simulink model "GRID_SUPPORTED_WIND_R1"  (R2026a)
settings: Solver=ode14x  StopTime=1.1  FixedStep=1e-5
InitFcn:
  | setup_v2_paths; init_grid_supported_integration;
undefined symbols (not defined in the file): Base, Control, Converter, Drive, Filter, PMSG, V2, Wind
libraries: nesl_utility x21, ee_lib x14, fl_lib x6, simulink x1
(part 1 of 2)
Description:
  | PV physical DC + optional corrected Wind R4 averaged GSC integration. The synchronous machine remains connected in every test. No BESS replacement or island certification.
settings Model: Creator=fakebob2004  LastModifiedBy=fakebob2004

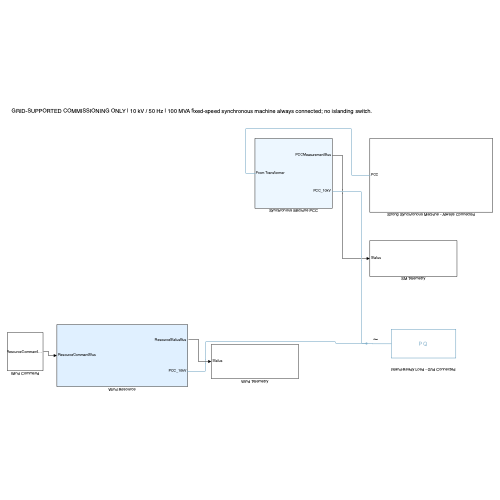
[thumbnail: Simulink's stored preview of the top-level diagram]
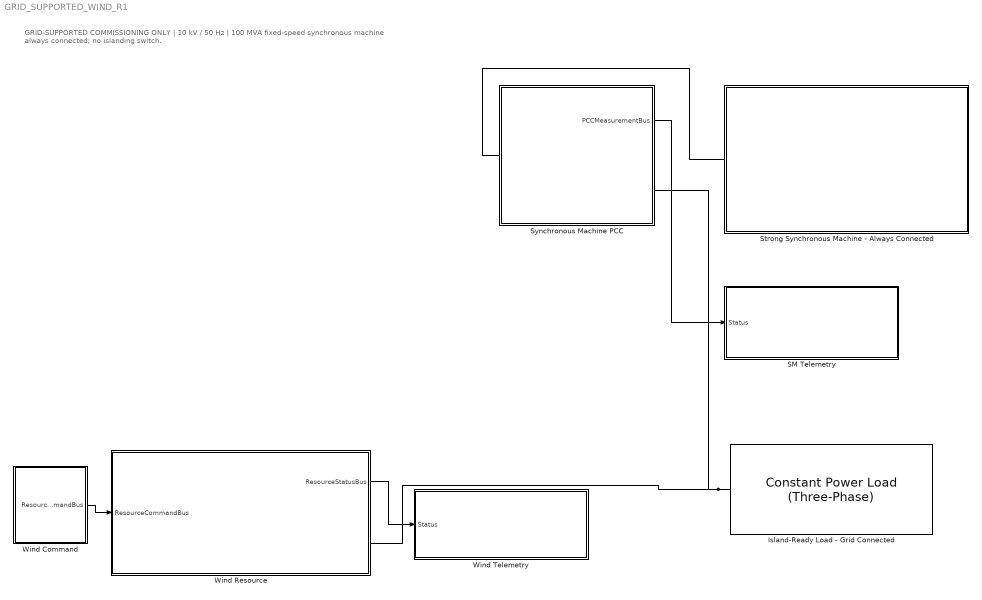
== system GRID_SUPPORTED_WIND_R1 ==
  note: GRID-SUPPORTED COMMISSIONING ONLY | 10 kV / 50 Hz | 100 MVA fixed-speed synchronous machine always connected; no islanding switch.
  Island-Ready Load - Grid Connected : ee_lib/Passive/Constant Power Load (Three-Phase)  port_option=ee.enum.threePhasePort.composite  FRated=50 Hz  active_power=5e6 W  reactive_power=1.5e6 V*A  Vline_rms_min=7000 V  tau=0.01 s  Vline_rms_ini=10000 V  Vang_ini=0 deg  gmin=1e-6 S
  SM Telemetry : Subsystem
  Strong Synchronous Machine - Always Connected : Subsystem
  Synchronous Machine PCC : Subsystem
  Wind Command : Subsystem
  Wind Resource : Subsystem
  Wind Telemetry : Subsystem
  wires:
  Synchronous Machine PCC/1(PCCMeasurementBus) -> SM Telemetry/1(Status)
  Wind Command/1(ResourceCommandBus) -> Wind Resource/1(ResourceCommandBus)
  Wind Resource/1(ResourceStatusBus) -> Wind Telemetry/1(Status)
  connections:
  Strong Synchronous Machine - Always Connected/LConn1 -- Synchronous Machine PCC/LConn1
  Synchronous Machine PCC/RConn1 -- Wind Resource/RConn1 -- Island-Ready Load - Grid Connected/LConn1

== system GRID_SUPPORTED_WIND_R1/SM Telemetry ==
  Status : Inport
  Fields : BusSelector  OutputSignals=P_W,Q_var,Vll_rms_V
  Record : ToWorkspace  VariableName=integration_sm  SaveFormat=Timeseries  SampleTime=-1
  Vector : Mux  Inputs=3
  wires:
  Status/1 -> Fields/1
  Fields/1 -> Vector/1  "<P_W>"
  Fields/2 -> Vector/2  "<Q_var>"
  Fields/3 -> Vector/3  "<Vll_rms_V>"
  Vector/1 -> Record/1

== system GRID_SUPPORTED_WIND_R1/Strong Synchronous Machine - Always Connected ==
  Excitation : Constant  Value=1e4*sqrt(2/3)
  Excitation PS : nesl_utility/Simulink-PS Converter  PhysicalDomain=network_engine_domain  SubClassName=ps_input  LeftPortType=input  RightPortType=output  PseudoPeriodic=off  Frequencies=[]  NoiseDistribution=none  NoiseParameters=[]  Unit=V  AffineConversion=off  FilteringAndDerivatives=zero  SimscapeFilterOrder=1  InputFilterTimeConstant=0.001  UdotUserProvided=0
  Governor Speed : Step  Time=10  InitialValue=2*pi*50  FinalValue=2*pi*50  SampleTime=0
  Ideal Governor : fl_lib/Mechanical/Mechanical Sources/Ideal Angular Velocity Source
  Machine Measurements : nesl_utility/PS-Simulink Converter  PhysicalDomain=network_engine_domain  SubClassName=ps_output  LeftPortType=input  RightPortType=output  PseudoPeriodic=off  Frequencies=[]  VectorFormat=inherit  Unit=1  AffineConversion=off
  Machine Record : ToWorkspace  VariableName=integration_machine  SaveFormat=Timeseries  SampleTime=-1
  Mechanical Reference : fl_lib/Mechanical/Rotational Elements/Mechanical Rotational Reference
  Neutral : fl_lib/Electrical/Electrical Elements/Electrical Reference
  Speed PS : nesl_utility/Simulink-PS Converter  PhysicalDomain=network_engine_domain  SubClassName=ps_input  LeftPortType=input  RightPortType=output  PseudoPeriodic=off  Frequencies=[]  NoiseDistribution=none  NoiseParameters=[]  Unit=rad/s  AffineConversion=off  FilteringAndDerivatives=zero  SimscapeFilterOrder=1  InputFilterTimeConstant=0.001  UdotUserProvided=0
  Synchronous Machine : ee_lib/Electromechanical/Synchronous/Simplified Synchronous Machine  port_option=ee.enum.threePhasePort.composite  SRated=100e6 A*V  VRated=10e3 V  FRated=50 Hz  nPolePairs=1  param_unit=ee.enum.unit.si  R_si=0.01 Ohm  L_si=0.001 H  R_pu=0.05  L_pu=0.3  initialization_option=ee.enum.sm.initialization.electrical  source_type=ee.enum.sm.load_flow_source_type.Swing  Vmag0=10e3 V  Vang0=0 deg  Pt0=5e6 A*V  Qt0=1.5e6 A*V  minimum_pu=0.95  phase_search_range=[-inf, inf] deg  gmin=1e-6 S  connection_option=ee.enum.Connection.wye  angular_position_diff_specify=off  angular_position_diff_priority=None  angular_position_diff=0 rad  angular_position_diff_nominal_specify=off  angular_position_diff_nominal_value=1  angular_position_diff_nominal_unit=rad  pu_psid_specify=off  pu_psid_priority=None  pu_psid=0  pu_psid_nominal_specify=off  pu_psid_nominal_value=1  pu_psid_nominal_unit=1  pu_psiq_specify=off  pu_psiq_priority=None  pu_psiq=0  pu_psiq_nominal_specify=off  pu_psiq_nominal_value=1  pu_psiq_nominal_unit=1  pu_psi0_specify=off  pu_psi0_priority=None  pu_psi0=0  pu_psi0_nominal_specify=off  pu_psi0_nominal_value=1  pu_psi0_nominal_unit=1  angular_torque_specify=off  angular_torque_priority=None  angular_torque=0 N*m  angular_torque_nominal_specify=off  angular_torque_nominal_value=1  angular_torque_nominal_unit=N*m  Tmeas=298.15 K  alpha=3.93e-3 1/K  stator_thermal_mass=100 J/K  rotor_thermal_mass=200 J/K  temperatureA_specify=off  temperatureA_priority=High  temperatureA=25 degC  temperatureA_nominal_specify=off  temperatureA_nominal_value=1  temperatureA_nominal_unit=degC  temperatureB_specify=off  temperatureB_priority=High  temperatureB=25 degC  temperatureB_nominal_specify=off  temperatureB_nominal_value=1  temperatureB_nominal_unit=degC  temperatureC_specify=off  temperatureC_priority=High  temperatureC=25 degC  temperatureC_nominal_specify=off  temperatureC_nominal_value=1  temperatureC_nominal_unit=degC  temperatureR_specify=off  temperatureR_priority=High  temperatureR=25 degC  temperatureR_nominal_specify=off  temperatureR_nominal_value=1  temperatureR_nominal_unit=degC
  PCC : PMIOPort  Side=Left  ConnectionType=Connection: foundation.electrical.three_phase
  wires:
  Machine Measurements/1 -> Machine Record/1
  Excitation/1 -> Excitation PS/1
  Governor Speed/1 -> Speed PS/1
  connections:
  Synchronous Machine/RConn1 -- Machine Measurements/LConn1
  Synchronous Machine/LConn3 -- Ideal Governor/RConn2 -- Mechanical Reference/LConn1
  Ideal Governor/LConn1 -- Synchronous Machine/LConn2
  Speed PS/RConn1 -- Ideal Governor/RConn1
  Excitation PS/RConn1 -- Synchronous Machine/LConn1
  Synchronous Machine/RConn3 -- Neutral/LConn1
  PCC/RConn1 -- Synchronous Machine/RConn2

== system GRID_SUPPORTED_WIND_R1/Synchronous Machine PCC ==
  Local PCC Voltage Record : ToWorkspace  VariableName=integration_bus_vabc  SaveFormat=Timeseries  SampleTime=-1
  Nominal Frequency : Constant  Value=V2.PV.rating.f_Hz
  P to Simulink : nesl_utility/PS-Simulink Converter  PhysicalDomain=network_engine_domain  SubClassName=ps_output  LeftPortType=input  RightPortType=output  PseudoPeriodic=off  Frequencies=[]  VectorFormat=inherit  Unit=W  AffineConversion=off
  PCC Measurement : BusCreator  Inputs=6  OutDataTypeStr=Bus: PCCMeasurementBus
  PCC Power Sensor : ee_lib/Sensors & Transducers/Power Sensor (Three-Phase)  port_option=ee.enum.threePhasePort.composite  load_type=ee.enum.passive.type_balanced.balanced  f0=60 Hz
  PCC VI Sensor : ee_lib/Sensors & Transducers/Current and Voltage Sensor (Three-Phase)  port_option=ee.enum.threePhasePort.composite  vMeasurementType=ee.enum.vmeasurement.ll  outputUnit=ee.enum.unit.si  SRated=100e6 A*V  VRated=24e3 V  I_specify=off  I_priority=None  I=[0, 0, 0] A  I_nominal_specify=off  I_nominal_value=1  I_nominal_unit=A  V_specify=off  V_priority=None  V=[0, 0, 0] V  V_nominal_specify=off  V_nominal_value=1  V_nominal_unit=V
  Q to Simulink : nesl_utility/PS-Simulink Converter  PhysicalDomain=network_engine_domain  SubClassName=ps_output  LeftPortType=input  RightPortType=output  PseudoPeriodic=off  Frequencies=[]  VectorFormat=inherit  Unit=W  AffineConversion=off
  Vll RMS : Fcn  Expr=sqrt((u(1)^2+u(2)^2+u(3)^2)/3)
  iabc to Simulink : nesl_utility/PS-Simulink Converter  PhysicalDomain=network_engine_domain  SubClassName=ps_output  LeftPortType=input  RightPortType=output  PseudoPeriodic=off  Frequencies=[]  VectorFormat=inherit  Unit=A  AffineConversion=off
  vabc to Simulink : nesl_utility/PS-Simulink Converter  PhysicalDomain=network_engine_domain  SubClassName=ps_output  LeftPortType=input  RightPortType=output  PseudoPeriodic=off  Frequencies=[]  VectorFormat=inherit  Unit=V  AffineConversion=off
  From Transformer : PMIOPort  Side=Left  ConnectionType=Connection: foundation.electrical.three_phase
  PCC_10kV : PMIOPort  Port=2  Side=Right  ConnectionType=Connection: foundation.electrical.three_phase
  PCCMeasurementBus : Outport  OutDataTypeStr=Bus: PCCMeasurementBus
  wires:
  vabc to Simulink/1 -> Vll RMS/1, Local PCC Voltage Record/1, PCC Measurement/1  "vabc_V"
  iabc to Simulink/1 -> PCC Measurement/2  "iabc_A"
  P to Simulink/1 -> PCC Measurement/3  "P_W"
  Q to Simulink/1 -> PCC Measurement/4  "Q_var"
  Vll RMS/1 -> PCC Measurement/5  "Vll_rms_V"
  Nominal Frequency/1 -> PCC Measurement/6  "frequency_Hz"
  PCC Measurement/1 -> PCCMeasurementBus/1
  connections:
  From Transformer/RConn1 -- PCC VI Sensor/LConn1
  PCC VI Sensor/RConn3 -- PCC Power Sensor/LConn1
  PCC Power Sensor/RConn1 -- PCC_10kV/RConn1
  PCC VI Sensor/RConn1 -- vabc to Simulink/LConn1
  PCC VI Sensor/RConn2 -- iabc to Simulink/LConn1
  PCC Power Sensor/LConn2 -- P to Simulink/LConn1
  PCC Power Sensor/LConn3 -- Q to Simulink/LConn1

== system GRID_SUPPORTED_WIND_R1/Wind Command ==
  Command : BusCreator  Inputs=6  OutDataTypeStr=Bus: ResourceCommandBus
  Enable : Constant
  Mode : Constant  Value=0
  P Base : Constant  Value=5000000
  P Increment : Step  Time=10  FinalValue=0  SampleTime=0
  P Reference : Sum
  Q Reference : Step  Time=10  FinalValue=0  SampleTime=0
  V Reference : Constant  Value=690
  f Reference : Constant  Value=50
  ResourceCommandBus : Outport  OutDataTypeStr=Bus: ResourceCommandBus
  wires:
  P Base/1 -> P Reference/1
  P Increment/1 -> P Reference/2
  P Reference/1 -> Command/1  "P_ref_W"
  Q Reference/1 -> Command/2  "Q_ref_var"
  V Reference/1 -> Command/3  "V_ref_V"
  f Reference/1 -> Command/4  "f_ref_Hz"
  Enable/1 -> Command/5  "enable"
  Mode/1 -> Command/6  "mode"
  Command/1 -> ResourceCommandBus/1

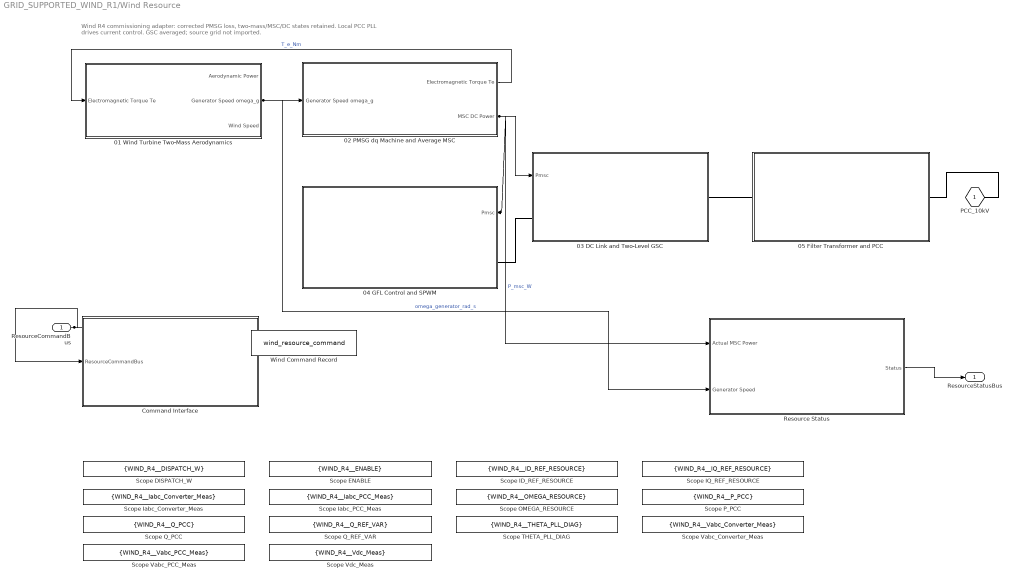
== system GRID_SUPPORTED_WIND_R1/Wind Resource ==
  note: Wind R4 commissioning adapter: corrected PMSG loss, two-mass/MSC/DC states retained. Local PCC PLL drives current control. GSC averaged; source grid not imported.
  ResourceCommandBus : Inport  OutDataTypeStr=Bus: ResourceCommandBus
  01 Wind Turbine Two-Mass Aerodynamics : Subsystem
  02 PMSG dq Machine and Average MSC : Subsystem
  03 DC Link and Two-Level GSC : Subsystem
  04 GFL Control and SPWM : Subsystem
      settings: PortSchema="{\"entries\":[{\"content\":{\"sides\":[{\"content\":{},\"type\":\"ConnectorPlacement.EquallySpacedRectSide\",\"uuid\":\"96295b0e-7f92-4eb5-94fb-1e379a07647e\"},{\"content\":{\"connectorIds\":[\"In1\",\"RConn1\"],\"side\":\"RIGHT\"},\"type\":\"ConnectorPlacement.EquallySpacedRectSide\",\"uuid\":\"831b7b8f-9668-4ddf-9feb-732f61fa57d8\"},{\"content\":{\"side\":\"TOP\"},\"type\":\"ConnectorPlacement.EquallySpacedRectSide\",\"uuid\":\"f19125e2-22e2-45e6-ab3f-ff5603225915\"},{\"content\":{\"side\":\"BOTTOM\"},\"type\":\"ConnectorPlacement.EquallySpacedRectSide\",\"uuid\":\"5342ef29-4f2f-4bd8-ad29-4f76b3f65d35\"}]},\"type\":\"ConnectorPlacement.EquallySpacedConnector\",\"uuid\":\"9af9a57b-5404-446b-bd5e-01cd06fadf4a\"}],\"packageUris\":[\"http://schema.mathworks.com/mf0/Connector/R2020b\"],\"version\":\"1.0\"}"
  05 Filter Transformer and PCC : Subsystem
  Command Interface : Subsystem
  Resource Status : Subsystem
  Scope DISPATCH_W : GotoTagVisibility  GotoTag=WIND_R4__DISPATCH_W
  Scope ENABLE : GotoTagVisibility  GotoTag=WIND_R4__ENABLE
  Scope ID_REF_RESOURCE : GotoTagVisibility  GotoTag=WIND_R4__ID_REF_RESOURCE
  Scope IQ_REF_RESOURCE : GotoTagVisibility  GotoTag=WIND_R4__IQ_REF_RESOURCE
  Scope Iabc_Converter_Meas : GotoTagVisibility  GotoTag=WIND_R4__Iabc_Converter_Meas
  Scope Iabc_PCC_Meas : GotoTagVisibility  GotoTag=WIND_R4__Iabc_PCC_Meas
  Scope OMEGA_RESOURCE : GotoTagVisibility  GotoTag=WIND_R4__OMEGA_RESOURCE
  Scope P_PCC : GotoTagVisibility  GotoTag=WIND_R4__P_PCC
  Scope Q_PCC : GotoTagVisibility  GotoTag=WIND_R4__Q_PCC
  Scope Q_REF_VAR : GotoTagVisibility  GotoTag=WIND_R4__Q_REF_VAR
  Scope THETA_PLL_DIAG : GotoTagVisibility  GotoTag=WIND_R4__THETA_PLL_DIAG
  Scope Vabc_Converter_Meas : GotoTagVisibility  GotoTag=WIND_R4__Vabc_Converter_Meas
  Scope Vabc_PCC_Meas : GotoTagVisibility  GotoTag=WIND_R4__Vabc_PCC_Meas
  Scope Vdc_Meas : GotoTagVisibility  GotoTag=WIND_R4__Vdc_Meas
  Wind Command Record : ToWorkspace  VariableName=wind_resource_command  SaveFormat=Timeseries  SampleTime=-1
  PCC_10kV : PMIOPort  Side=Right  ConnectionType=Connection: foundation.electrical.three_phase
  ResourceStatusBus : Outport  OutDataTypeStr=Bus: ResourceStatusBus
  wires:
  01 Wind Turbine Two-Mass Aerodynamics/2(Generator Speed omega_g) -> 02 PMSG dq Machine and Average MSC/1(Generator Speed omega_g), Resource Status/2(Generator Speed)  "omega_generator_rad_s"
  02 PMSG dq Machine and Average MSC/1(Electromagnetic Torque Te) -> 01 Wind Turbine Two-Mass Aerodynamics/1(Electromagnetic Torque Te)  "T_e_Nm"
  02 PMSG dq Machine and Average MSC/2(MSC DC Power) -> 03 DC Link and Two-Level GSC/1(Pmsc), 04 GFL Control and SPWM/1(Pmsc), Resource Status/1(Actual MSC Power)  "P_msc_W"
  ResourceCommandBus/1 -> Command Interface/1(ResourceCommandBus), Wind Command Record/1
  Resource Status/1(Status) -> ResourceStatusBus/1
  connections:
  04 GFL Control and SPWM/RConn1 -- 03 DC Link and Two-Level GSC/LConn1
  03 DC Link and Two-Level GSC/RConn1 -- 05 Filter Transformer and PCC/LConn1
  05 Filter Transformer and PCC/RConn1 -- PCC_10kV/RConn1

== system GRID_SUPPORTED_WIND_R1/Wind Telemetry ==
  Status : Inport
  Fields : BusSelector  OutputSignals=P_W,Q_var,Vpcc_V,frequency_Hz,available_power_W,power_headroom_W,current_limit_factor,energy_state_pu,Vdc_V,control_mode,healthy
  Record : ToWorkspace  VariableName=integration_wind  SaveFormat=Timeseries  SampleTime=-1
  Vector : Mux  Inputs=11
  wires:
  Status/1 -> Fields/1
  Fields/1 -> Vector/1  "<P_W>"
  Fields/2 -> Vector/2  "<Q_var>"
  Fields/3 -> Vector/3  "<Vpcc_V>"
  Fields/4 -> Vector/4  "<frequency_Hz>"
  Fields/5 -> Vector/5  "<available_power_W>"
  Fields/6 -> Vector/6  "<power_headroom_W>"
  Fields/7 -> Vector/7  "<current_limit_factor>"
  Fields/8 -> Vector/8  "<energy_state_pu>"
  Fields/9 -> Vector/9  "<Vdc_V>"
  Fields/10 -> Vector/10  "<control_mode>"
  Fields/11 -> Vector/11  "<healthy>"
  Vector/1 -> Record/1

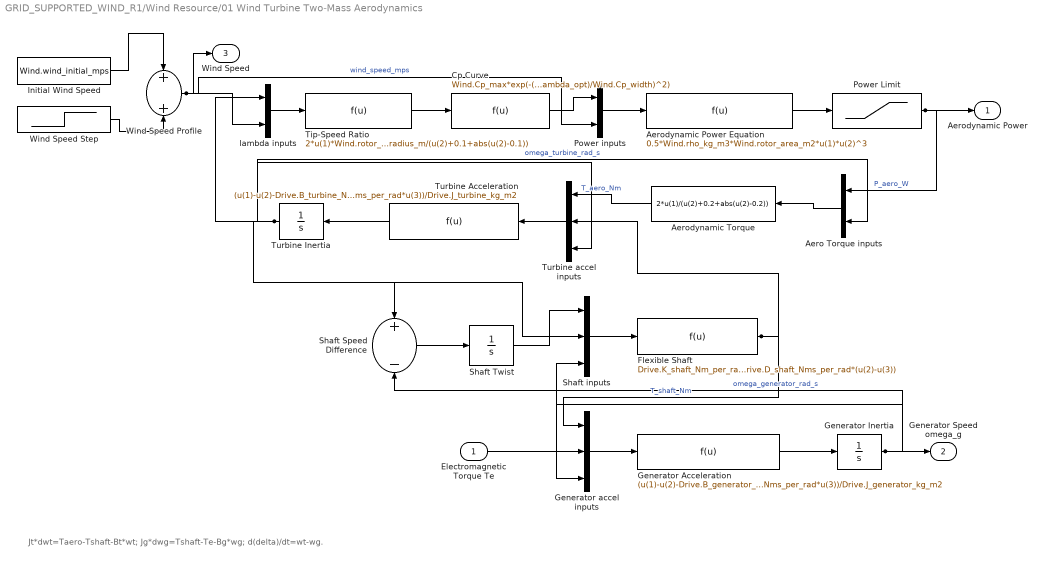
== system GRID_SUPPORTED_WIND_R1/Wind Resource/01 Wind Turbine Two-Mass Aerodynamics ==
  note: Jt*dwt=Taero-Tshaft-Bt*wt; Jg*dwg=Tshaft-Te-Bg*wg; d(delta)/dt=wt-wg.
  Electromagnetic Torque Te : Inport
  Aero Torque inputs : Mux  Inputs=2
  Aerodynamic Power Equation : Fcn  Expr=0.5*Wind.rho_kg_m3*Wind.rotor_area_m2*u(1)*u(2)^3
  Aerodynamic Torque : Fcn  Expr=2*u(1)/(u(2)+0.2+abs(u(2)-0.2))
  Cp Curve : Fcn  Expr=Wind.Cp_max*exp(-((u-Wind.lambda_opt)/Wind.Cp_width)^2)
  Flexible Shaft : Fcn  Expr=Drive.K_shaft_Nm_per_rad*u(1)+Drive.D_shaft_Nms_per_rad*(u(2)-u(3))
  Generator Acceleration : Fcn  Expr=(u(1)-u(2)-Drive.B_generator_Nms_per_rad*u(3))/Drive.J_generator_kg_m2
  Generator Inertia : Integrator  InitialCondition=PMSG.Init.omega_rad_s
  Generator accel inputs : Mux  Inputs=3
  Initial Wind Speed : Constant  Value=Wind.wind_initial_mps
  Power Limit : Saturate  UpperLimit=1.10*Wind.P_rated_W  LowerLimit=0
  Power inputs : Mux  Inputs=2
  Shaft Speed Difference : Sum  Inputs=+-
  Shaft Twist : Integrator  InitialCondition=PMSG.Init.shaft_angle_rad
  Shaft inputs : Mux  Inputs=3
  Tip-Speed Ratio : Fcn  Expr=2*u(1)*Wind.rotor_radius_m/(u(2)+0.1+abs(u(2)-0.1))
  Turbine Acceleration : Fcn  Expr=(u(1)-u(2)-Drive.B_turbine_Nms_per_rad*u(3))/Drive.J_turbine_kg_m2
  Turbine Inertia : Integrator  InitialCondition=PMSG.Init.omega_rad_s
  Turbine accel inputs : Mux  Inputs=3
  Wind Speed Profile : Sum
  Wind Speed Step : Step  Time=0.75  FinalValue=Wind.wind_step_mps  SampleTime=0
  lambda inputs : Mux  Inputs=2
  Aerodynamic Power : Outport
  Generator Speed omega_g : Outport  Port=2
  Wind Speed : Outport  Port=3
  wires:
  Shaft inputs/1 -> Flexible Shaft/1
  Shaft Twist/1 -> Shaft inputs/1
  Shaft Speed Difference/1 -> Shaft Twist/1
  Generator Acceleration/1 -> Generator Inertia/1
  Generator accel inputs/1 -> Generator Acceleration/1
  Generator Inertia/1 -> Generator Speed omega_g/1, Shaft inputs/3, Shaft Speed Difference/2, Generator accel inputs/3  "omega_generator_rad_s"
  Electromagnetic Torque Te/1 -> Generator accel inputs/2
  Turbine Acceleration/1 -> Turbine Inertia/1
  Turbine accel inputs/1 -> Turbine Acceleration/1
  Flexible Shaft/1 -> Generator accel inputs/1, Turbine accel inputs/2  "T_shaft_Nm"
  Aerodynamic Torque/1 -> Turbine accel inputs/1  "T_aero_Nm"
  Aero Torque inputs/1 -> Aerodynamic Torque/1
  Power Limit/1 -> Aero Torque inputs/1, Aerodynamic Power/1  "P_aero_W"
  Aerodynamic Power Equation/1 -> Power Limit/1
  Power inputs/1 -> Aerodynamic Power Equation/1
  Cp Curve/1 -> Power inputs/1
  Tip-Speed Ratio/1 -> Cp Curve/1
  lambda inputs/1 -> Tip-Speed Ratio/1
  Turbine Inertia/1 -> Shaft inputs/2, Shaft Speed Difference/1, Turbine accel inputs/3, Aero Torque inputs/2, lambda inputs/1  "omega_turbine_rad_s"
  Wind Speed Profile/1 -> Power inputs/2, lambda inputs/2, Wind Speed/1  "wind_speed_mps"
  Wind Speed Step/1 -> Wind Speed Profile/2
  Initial Wind Speed/1 -> Wind Speed Profile/1

== system GRID_SUPPORTED_WIND_R1/Wind Resource/02 PMSG dq Machine and Average MSC ==
  note: dq convention: generating iq < 0 and Te > 0. Voltage commands include cross-coupling and back-EMF feedforward plus circular Vdc limit.
  Generator Speed omega_g : Inport
  01 Torque and Current References : Subsystem
  02 MSC Current Control : Subsystem
  03 PMSG Electrical Dynamics : Subsystem
  04 MSC DC Power : Subsystem
  Electrical Speed : Gain  Gain=PMSG.pole_pairs
  Electromagnetic Torque Te : Outport
  MSC DC Power : Outport  Port=2
  wires:
  04 MSC DC Power/1(Pdc) -> MSC DC Power/1
  03 PMSG Electrical Dynamics/1(Te) -> Electromagnetic Torque Te/1
  02 MSC Current Control/2(vq) -> 04 MSC DC Power/2(vq), 03 PMSG Electrical Dynamics/2(vq)
  02 MSC Current Control/1(vd) -> 04 MSC DC Power/1(vd), 03 PMSG Electrical Dynamics/1(vd)
  03 PMSG Electrical Dynamics/3(iq) -> 04 MSC DC Power/4(iq), 02 MSC Current Control/5(iq)
  03 PMSG Electrical Dynamics/2(id) -> 04 MSC DC Power/3(id), 02 MSC Current Control/4(id)
  Electrical Speed/1 -> 03 PMSG Electrical Dynamics/3(omega_e), 02 MSC Current Control/3(omega_e)
  01 Torque and Current References/2(iq_ref) -> 02 MSC Current Control/2(iq_ref)
  01 Torque and Current References/1(id_ref) -> 02 MSC Current Control/1(id_ref)
  Generator Speed omega_g/1 -> 01 Torque and Current References/1(omega_g), Electrical Speed/1

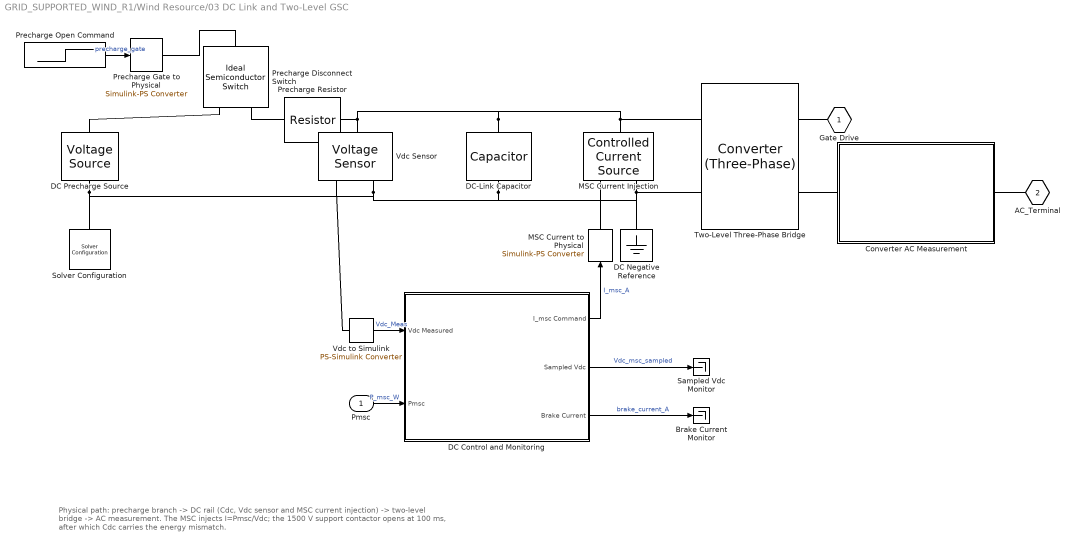
== system GRID_SUPPORTED_WIND_R1/Wind Resource/03 DC Link and Two-Level GSC ==
  note: Physical path: precharge branch -> DC rail (Cdc, Vdc sensor and MSC current injection) -> two-level bridge -> AC measurement.
      | The MSC injects I=Pmsc/Vdc; the 1500 V support contactor opens at 100 ms, after which Cdc carries the energy mismatch.
  Pmsc : Inport
  Brake Current Monitor : Terminator
  Converter AC Measurement : Subsystem
  DC Control and Monitoring : Subsystem
  DC Negative Reference : fl_lib/Electrical/Electrical Elements/Electrical Reference
  DC Precharge Source : ee_lib/Sources/Voltage Source  dc_voltage=Converter.Vdc_nom V  ac_voltage=0 V  ac_shift=0 rad  ac_frequency=60 Hz  noise_mode=ee.enum.sources.noise.Disabled  PSD=0 V^2/Hz  sample_time=1e-3 s  repeatability=ee.enum.sources.repeatability.NotRepeatable  user_seed=0  auto_seed=3499211588  i_specify=off  i_priority=None  i=0 A  i_nominal_specify=off  i_nominal_value=1  i_nominal_unit=A  v_specify=off  v_priority=None  v=0 V  v_nominal_specify=off  v_nominal_value=1  v_nominal_unit=V
  DC-Link Capacitor : ee_lib/Passive/Capacitor  cap_option=ee.enum.passive.capacitor.capOption.const  c=Converter.Cdc F  Cvec=[1e-05, 1e-06] F  Vvec=[0, 10] V  CV_table_symmetry=ee.enum.passive.capacitor.tableSymmetry.yes  f_vec=[1, 10] kHz  DFext_vec=[.8, 1.2]  enable_C_tol=ee.enum.toleranceApplication.none  averaging_period=0 s  C_tol=5  tol_distribution=ee.enum.toleranceDistribution.uniform  nSigma=4  r=Converter.Cdc_esr Ohm  g=0 1/Ohm  enable_operating_limits=ee.enum.enable.no  operating_limit_action=ee.enum.passive.reportOpLim.warn  max_working_voltage_range=[-25, 25] V  power_rating=1 W  maxTemperature=85 degC  thermalEnable=false  thermalMass=1 J/K  i_specify=off  i_priority=None  i=0 A  i_nominal_specify=off  i_nominal_value=1  i_nominal_unit=A  v_specify=on  v_priority=High  v=Converter.Vdc_nom V  v_nominal_specify=off  v_nominal_value=1  v_nominal_unit=V  vc_specify=off  vc_priority=High  vc=0 V  vc_nominal_specify=off  vc_nominal_value=1  vc_nominal_unit=V  T_specify=off  T_priority=None  T=298.15 K  T_nominal_specify=off  T_nominal_value=1  T_nominal_unit=K
  MSC Current Injection : fl_lib/Electrical/Electrical Sources/Controlled Current Source
  MSC Current to Physical : nesl_utility/Simulink-PS Converter  PhysicalDomain=network_engine_domain  SubClassName=ps_input  LeftPortType=input  RightPortType=output  PseudoPeriodic=off  Frequencies=[]  NoiseDistribution=none  NoiseParameters=[]  Unit=A  AffineConversion=off  FilteringAndDerivatives=provide  SimscapeFilterOrder=1  InputFilterTimeConstant=0.001  UdotUserProvided=0
  Precharge Disconnect Switch : ee_lib/Semiconductors & Converters/Ideal Semiconductor Switch  port_option=ee.enum.controlport.ps  Ron=Wind.brake_switch_Ron_ohm Ohm  Goff=Wind.brake_switch_Goff_S 1/Ohm  Vth=0.5 V  diode_param=ee.enum.semiconductors.protectionDiode.external  diode_Vf=0.8 V  diode_Ron=0.001 Ohm  diode_Goff=1e-5 1/Ohm  diode_C=50e-9 F  diode_iRM=-235 A  diode_iF=300 A  diode_idot=-50 A/us  diode_trr_param=ee.enum.converters.diodetrr.trr_factor  diode_trr_factor=3  diode_trr=15 us  diode_Qrr=1500 s*uA
  Precharge Gate to Physical : nesl_utility/Simulink-PS Converter  PhysicalDomain=network_engine_domain  SubClassName=ps_input  LeftPortType=input  RightPortType=output  PseudoPeriodic=off  Frequencies=[]  NoiseDistribution=none  NoiseParameters=[]  Unit=1  AffineConversion=off  FilteringAndDerivatives=provide  SimscapeFilterOrder=1  InputFilterTimeConstant=0.001  UdotUserProvided=0
  Precharge Open Command : Step  Time=Wind.precharge_open_time_s  InitialValue=1  FinalValue=0  SampleTime=0
  Precharge Resistor : ee_lib/Passive/Resistor  R=Wind.precharge_R_ohm Ohm  enable_R_tol=ee.enum.toleranceApplication.none  R_tol=5  tol_distribution=ee.enum.toleranceDistribution.uniform  nSigma=4  enable_operating_limits=ee.enum.enable.no  operating_limit_action=ee.enum.passive.reportOpLim.warn  power_rating=1 W  max_working_voltage=100 V  noise_mode=ee.enum.sources.noise.Disabled  Tdevice=25 degC  sample_time=1e-3 s  repeatability=ee.enum.ic.repeatability.notRepeatable  user_seed=0  auto_seed=3890346746  power_derating_T1=70 degC  power_derating_T2=155 degC  operating_temperature_range_vec=[-50, 150] degC  alpha=3.93e-3 1/K  Tmeas=25 degC  thermal_mass=100 J/K  temperature_specify=off  temperature_priority=High  temperature=298.15 K  temperature_nominal_specify=off  temperature_nominal_value=1  temperature_nominal_unit=K
  Sampled Vdc Monitor : Terminator
  Solver Configuration : nesl_utility/Solver Configuration  PhysicalDomain=network_engine_domain  SubClassName=solver  LeftPortType=input  RightPortType=generic  Tones=[]  Harmonics=[]  SimulateNoise=off  Profile=off  UseLocalSampling=off  EnableSwitchedLinearOptims=on  FrequencyDomain=off  UseCCode=off  RelTol=0.001  AbsTol=0.001  MinStep=1e-09  ToWorkspace=off  RevertToSquareIcSolve=off  NumHomotopyIterations=100  PhasorMode=off  PhasorModeNumHarmonics=1  ConsistencySolver=NEWTON_XTOL_AFTER_FTOL  CanonicalOrdering=CANONICAL  OptimizeIntermediates=OPTIMIZED  IndexReductionMethod=DerivativeReplacement  DoDC=off  ResidualTolerance=1e-09  ConsistencyTolSource=GLOBAL  ConsistencyAbsTol=0.001  ConsistencyRelTol=0.001  ConsistencyTolFactor=0.001  UseLocalSolver=off  LocalSolverChoice=NE_BACKWARD_EULER_ADVANCER  ResolveIndetEquations=on  FunctionEvalNumThread=1  LocalSolverSampleTime=0.001  DoFixedCost=off  MaxNonlinIter=3  MaxModeIter=2  ComputeImpulses=off  ImpulseIterations=2  LinearAlgebra=auto  LinearAlgebraNumThread=0  EquationFormulation=NE_TIME_EF  DelaysMemoryBudget=1024  AutomaticFiltering=on  FilteringTimeConstant=0.001  PartitionStorageMethod=AS_NEEDED  PartitionMemoryBudget=1024  PartitionMethod=ROBUST  MultibodyUseLocalSolver=off  MultibodyLocalSolverChoice=ODE1  MultibodyLocalSolverSampleTime=0.001
  Two-Level Three-Phase Bridge : ee_lib/Semiconductors & Converters/Converters/Converter (Three-Phase)  port_option=ee.enum.threePhasePort.composite  fidelity_option=ee.enum.converters.fidelity.detailed  device_type=ee.enum.converters.switchingdevice.averaged  showThermalPort=false  K=0  Vth=Converter.GateThresholdVoltage V  Vgt=1 V  Vgt_off=-1 V  Ih=1 A  Vf=0.8 V  Ron=Converter.SwitchOnResistance Ohm  Rds=0.001 Ohm  Goff=Converter.OffConductance 1/Ohm  Eon_scalar=22.86e-3 J  Eoff_scalar=17.14e-3 J  Eoff_natural_commutation=10e-3 J  Voff=300 V  Iout_scalar=600 A  onCurrentMeasDelay=0 s  useCurrentFromPreviousCycle=false  useVoltageFromPreviousCycle=false  diode_param=ee.enum.converters.protectiondiode.nodynamics  diode_Vf=0.8 V  diode_Ron=0.001 Ohm  diode_Goff=1e-5 1/Ohm  diode_C=50 nF  diode_iRM=-235 A  diode_iF=300 A  diode_idot=-50 A/us  diode_trr_param=ee.enum.converters.diodetrr.trr_factor  diode_trr_factor=3  diode_trr=15 us  diode_Qrr=1500 s*uA  diode_rec_loss_model=ee.enum.diode.reverseRecoveryModel.fixed  diode_ErecVal=0 J  diode_scaleWithIandV=false  diode_ErecMat=zeros(2, 3) J  diode_TjrecVec=[298.15, 398.15] K  diode_IfrecVec=[.1, 1, 10] A  diode_IrecVal=10 A  diode_VrecVal=10 V  diode_tFilter=1 / 1000 / 100 s  thermal_network_parameterization=ee.enum.thermalNetworkTopology.external  Rth=[.08, .5] K/W  Rth_Cauer=[.08, .1, .5] K/W  Rth_Foster=[.08, .14, .22, .16] K/W  thermal_mass_parameterization=ee.enum.thermalNetwork.timeconstant  thermal_mass=[.01, .5] J/K  thermal_mass_Cauer=[.01, .1, .5] J/K  thermal_mass_Foster=[.001, .005, .05, .5] J/K  thermal_time_constant=[.001, .2] s  thermal_time_constant_Cauer=[.001, .1, .2] s  thermal_time_constant_Foster=[7e-05, .0007, .01, .08] s  thermal_mass_initial_temperatures=[25, 25] degC  thermal_mass_initial_temperatures_Cauer=[25, 25, 25] degC  junction_thermal_mass=0.01 J/K  Tvec_initial_Foster=[25, 25, 25, 25] degC  snubber_type=ee.enum.converters.snubber.exclude  Cs=1e-7 F  Rs=0.1 Ohm  Vce_loss=[0, 150, 300] V
  Vdc Sensor : fl_lib/Electrical/Electrical Sensors/Voltage Sensor
  Vdc to Simulink : nesl_utility/PS-Simulink Converter  PhysicalDomain=network_engine_domain  SubClassName=ps_output  LeftPortType=input  RightPortType=output  PseudoPeriodic=off  Frequencies=[]  VectorFormat=inherit  Unit=V  AffineConversion=off
  Gate Drive : PMIOPort  Side=Left
  AC_Terminal : PMIOPort  Port=2  Side=Right
  wires:
  Precharge Open Command/1 -> Precharge Gate to Physical/1  "precharge_gate"
  DC Control and Monitoring/3(Brake Current) -> Brake Current Monitor/1  "brake_current_A"
  DC Control and Monitoring/2(Sampled Vdc) -> Sampled Vdc Monitor/1  "Vdc_msc_sampled"
  DC Control and Monitoring/1(I_msc Command) -> MSC Current to Physical/1  "I_msc_A"
  Pmsc/1 -> DC Control and Monitoring/2(Pmsc)  "P_msc_W"
  Vdc to Simulink/1 -> DC Control and Monitoring/1(Vdc Measured)  "Vdc_Meas"
  connections:
  Precharge Gate to Physical/RConn1 -- Precharge Disconnect Switch/LConn1
  DC Negative Reference/LConn1 -- MSC Current Injection/RConn2 -- Two-Level Three-Phase Bridge/RConn2 -- DC-Link Capacitor/RConn1 -- Solver Configuration/RConn1 -- DC Precharge Source/RConn1 -- Vdc Sensor/RConn2
  Two-Level Three-Phase Bridge/RConn1 -- MSC Current Injection/LConn1 -- DC-Link Capacitor/LConn1 -- Precharge Resistor/RConn1 -- Vdc Sensor/LConn1
  Precharge Disconnect Switch/RConn2 -- Precharge Resistor/LConn1
  DC Precharge Source/LConn1 -- Precharge Disconnect Switch/RConn1
  MSC Current to Physical/RConn1 -- MSC Current Injection/RConn1
  Converter AC Measurement/RConn1 -- AC_Terminal/RConn1
  Two-Level Three-Phase Bridge/LConn2 -- Converter AC Measurement/LConn1
  Vdc Sensor/RConn1 -- Vdc to Simulink/LConn1
  Gate Drive/RConn1 -- Two-Level Three-Phase Bridge/LConn1

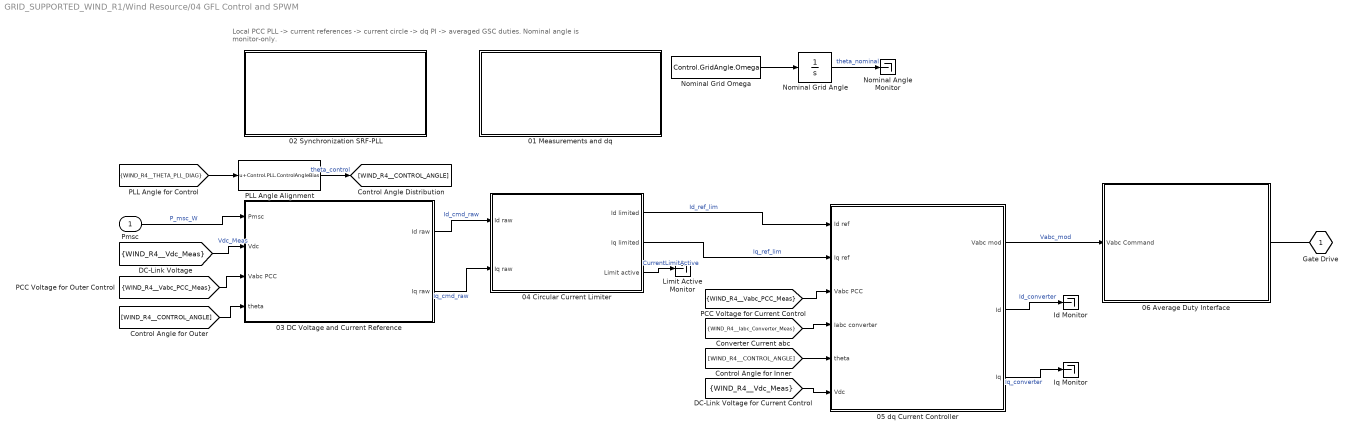
== system GRID_SUPPORTED_WIND_R1/Wind Resource/04 GFL Control and SPWM ==
  note: Local PCC PLL -> current references -> current circle -> dq PI -> averaged GSC duties. Nominal angle is monitor-only.
  Pmsc : Inport
  01 Measurements and dq : Subsystem
  02 Synchronization SRF-PLL : Subsystem
  03 DC Voltage and Current Reference : Subsystem
  04 Circular Current Limiter : Subsystem
  05 dq Current Controller : Subsystem
  06 Average Duty Interface : Subsystem
  Id Monitor : Terminator
  Iq Monitor : Terminator
  Limit Active Monitor : Terminator
  Nominal Angle Monitor : Terminator
  Nominal Grid Angle : Integrator  InitialCondition=Control.GridAngle.Theta0
  Nominal Grid Omega : Constant  Value=Control.GridAngle.Omega
  PLL Angle Alignment : Bias  Bias=Control.PLL.ControlAngleBias  SaturateOnIntegerOverflow=off
  Gate Drive : PMIOPort  Side=Right
  wires:
  Nominal Grid Angle/1 -> Nominal Angle Monitor/1  "theta_nominal"
  04 Circular Current Limiter/3(Limit active) -> Limit Active Monitor/1  "CurrentLimitActive"
  05 dq Current Controller/3(Iq) -> Iq Monitor/1  "Iq_converter"
  05 dq Current Controller/2(Id) -> Id Monitor/1  "Id_converter"
  [WIND_R4__Vdc_Meas] -> 05 dq Current Controller/6(Vdc)
  [WIND_R4__CONTROL_ANGLE] -> 05 dq Current Controller/5(theta)
  [WIND_R4__Iabc_Converter_Meas] -> 05 dq Current Controller/4(Iabc converter)
  [WIND_R4__Vabc_PCC_Meas] -> 05 dq Current Controller/3(Vabc PCC)
  04 Circular Current Limiter/2(Iq limited) -> 05 dq Current Controller/2(Iq ref)  "Iq_ref_lim"
  04 Circular Current Limiter/1(Id limited) -> 05 dq Current Controller/1(Id ref)  "Id_ref_lim"
  03 DC Voltage and Current Reference/2(Iq raw) -> 04 Circular Current Limiter/2(Iq raw)  "Iq_cmd_raw"
  03 DC Voltage and Current Reference/1(Id raw) -> 04 Circular Current Limiter/1(Id raw)  "Id_cmd_raw"
  [WIND_R4__CONTROL_ANGLE] -> 03 DC Voltage and Current Reference/4(theta)
  PLL Angle Alignment/1 -> [WIND_R4__CONTROL_ANGLE]  "theta_control"
  Nominal Grid Omega/1 -> Nominal Grid Angle/1
  [WIND_R4__Vabc_PCC_Meas] -> 03 DC Voltage and Current Reference/3(Vabc PCC)
  [WIND_R4__Vdc_Meas] -> 03 DC Voltage and Current Reference/2(Vdc)  "Vdc_Meas"
  Pmsc/1 -> 03 DC Voltage and Current Reference/1(Pmsc)  "P_msc_W"
  05 dq Current Controller/1(Vabc mod) -> 06 Average Duty Interface/1(Vabc Command)  "Vabc_mod"
  [WIND_R4__THETA_PLL_DIAG] -> PLL Angle Alignment/1
  connections:
  06 Average Duty Interface/RConn1 -- Gate Drive/RConn1

== system GRID_SUPPORTED_WIND_R1/Wind Resource/05 Filter Transformer and PCC ==
  note: Direct power path: Rf + Lf -> 0.69/10 kV Y-Y transformer -> PCC VI sensor. Measurements remain internal and logged.
  0.69 kV to 10 kV Step-Up Transformer : ee_lib/Passive/Transformers/Two-Winding Transformer (Three-Phase)  SRated=Transformer.Sn A*V  FRated=Transformer.f Hz  Winding1Connection=ee.enum.windingconnection.Y  VRated1=Transformer.Vll_primary V  Winding2Connection=ee.enum.windingconnection.Y  VRated2=Transformer.Vll_secondary V  CoreType=ee.enum.coretype.threelimb  pu_Rw1=Transformer.R1_pu  pu_Rw2=Transformer.R2_pu  leakage_reactance_option=ee.enum.transformer_leakage.exclude  pu_Xl1=Transformer.X1_pu  pu_Xl2=Transformer.X2_pu  magnetizing_resistance_option=ee.enum.transformer_magnetizingResistance.exclude  pu_Rm=500  magnetizing_reactance_option=ee.enum.transformer_magnetizingReactance.exclude  saturation_option=ee.enum.transformer_saturation.exclude  pu_Xm=Transformer.Xm_pu  current_data=[0, .002, 1, 2]  magnetic_flux_data=[0, 1.2, 1.5, 1.51]  pu_X0=0.5  i1_specify=off  i1_priority=None  i1=[0, 0, 0] A  i1_nominal_specify=off  i1_nominal_value=1  i1_nominal_unit=A  i2_specify=off  i2_priority=None  i2=[0, 0, 0] A  i2_nominal_specify=off  i2_nominal_value=1  i2_nominal_unit=A  phi_specify=off  phi_priority=None  phi=[0, 0, 0]  phi_nominal_specify=off  phi_nominal_value=1  phi_nominal_unit=1
  AC Filter Rf + Lf : ee_lib/Passive/RLC Assemblies/RLC (Three-Phase)  port_option=ee.enum.threePhasePort.composite  component_structure=ee.enum.rlc.structure.SeriesRL  R=Filter.R Ohm  L=Filter.L H  C=1e-6 F  R_parasitic=0 Ohm  G_parasitic=0 1/Ohm  IL_specify=off  IL_priority=High  IL=[0, 0, 0] A  IL_nominal_specify=off  IL_nominal_value=1  IL_nominal_unit=A  VC_specify=off  VC_priority=High  VC=[0, 0, 0] V  VC_nominal_specify=off  VC_nominal_value=1  VC_nominal_unit=V
  Iabc PCC to Simulink : nesl_utility/PS-Simulink Converter  PhysicalDomain=network_engine_domain  SubClassName=ps_output  LeftPortType=input  RightPortType=output  PseudoPeriodic=off  Frequencies=[]  VectorFormat=inherit  Unit=A  AffineConversion=off
  PCC VI Sensor : ee_lib/Sensors & Transducers/Current and Voltage Sensor (Three-Phase)  port_option=ee.enum.threePhasePort.composite  vMeasurementType=ee.enum.vmeasurement.lg  outputUnit=ee.enum.unit.si  SRated=Base.Sn A*V  VRated=Base.Vll_hv V  I_specify=off  I_priority=None  I=[0, 0, 0] A  I_nominal_specify=off  I_nominal_value=1  I_nominal_unit=A  V_specify=off  V_priority=None  V=[0, 0, 0] V  V_nominal_specify=off  V_nominal_value=1  V_nominal_unit=V
  Vabc PCC to Simulink : nesl_utility/PS-Simulink Converter  PhysicalDomain=network_engine_domain  SubClassName=ps_output  LeftPortType=input  RightPortType=output  PseudoPeriodic=off  Frequencies=[]  VectorFormat=inherit  Unit=V  AffineConversion=off
  From_VSC : PMIOPort  Side=Left
  To_Grid : PMIOPort  Port=2  Side=Right
  tag scope: WIND_R4__Iabc_PCC_Meas=scoped, WIND_R4__Vabc_PCC_Meas=scoped
  wires:
  Iabc PCC to Simulink/1 -> [WIND_R4__Iabc_PCC_Meas]  "Iabc_PCC_Meas"
  Vabc PCC to Simulink/1 -> [WIND_R4__Vabc_PCC_Meas]  "Vabc_PCC_Meas"
  connections:
  PCC VI Sensor/RConn2 -- Iabc PCC to Simulink/LConn1
  PCC VI Sensor/RConn1 -- Vabc PCC to Simulink/LConn1
  PCC VI Sensor/RConn3 -- To_Grid/RConn1
  0.69 kV to 10 kV Step-Up Transformer/RConn1 -- PCC VI Sensor/LConn1
  AC Filter Rf + Lf/RConn1 -- 0.69 kV to 10 kV Step-Up Transformer/LConn1
  From_VSC/RConn1 -- AC Filter Rf + Lf/LConn1

== system GRID_SUPPORTED_WIND_R1/Wind Resource/Command Interface ==
  ResourceCommandBus : Inport  OutDataTypeStr=Bus: ResourceCommandBus
  Command Selector : BusSelector  OutputSignals=P_ref_W,Q_ref_var,enable
  tag scope: WIND_R4__DISPATCH_W=scoped, WIND_R4__ENABLE=scoped, WIND_R4__Q_REF_VAR=scoped
  wires:
  ResourceCommandBus/1 -> Command Selector/1
  Command Selector/1 -> [WIND_R4__DISPATCH_W]  "<P_ref_W>"
  Command Selector/2 -> [WIND_R4__Q_REF_VAR]  "<Q_ref_var>"
  Command Selector/3 -> [WIND_R4__ENABLE]  "<enable>"

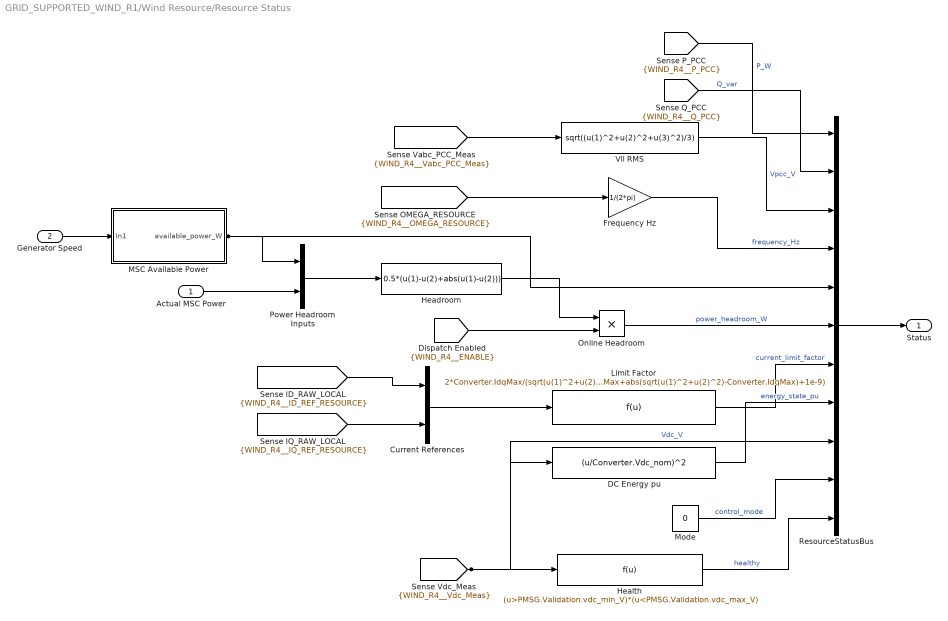
== system GRID_SUPPORTED_WIND_R1/Wind Resource/Resource Status ==
  Actual MSC Power : Inport
  Generator Speed : Inport  Port=2
  Current References : Mux  Inputs=2
  DC Energy pu : Fcn  Expr=(u/Converter.Vdc_nom)^2
  Frequency Hz : Gain  Gain=1/(2*pi)
  Headroom : Fcn  Expr=0.5*(u(1)-u(2)+abs(u(1)-u(2)))
  Health : Fcn  Expr=(u>PMSG.Validation.vdc_min_V)*(u<PMSG.Validation.vdc_max_V)
  Limit Factor : Fcn  Expr=2*Converter.IdqMax/(sqrt(u(1)^2+u(2)^2)+Converter.IdqMax+abs(sqrt(u(1)^2+u(2)^2)-Converter.IdqMax)+1e-9)
  MSC Available Power : Subsystem
  Mode : Constant  Value=0
  Online Headroom : Product
  Power Headroom Inputs : Mux  Inputs=2
  ResourceStatusBus : BusCreator  Inputs=11  OutDataTypeStr=Bus: ResourceStatusBus
  Vll RMS : Fcn  Expr=sqrt((u(1)^2+u(2)^2+u(3)^2)/3)
  Status : Outport  OutDataTypeStr=Bus: ResourceStatusBus
  wires:
  DC Energy pu/1 -> ResourceStatusBus/8  "energy_state_pu"
  Limit Factor/1 -> ResourceStatusBus/7  "current_limit_factor"
  ResourceStatusBus/1 -> Status/1
  Online Headroom/1 -> ResourceStatusBus/6  "power_headroom_W"
  Vll RMS/1 -> ResourceStatusBus/3  "Vpcc_V"
  Mode/1 -> ResourceStatusBus/10  "control_mode"
  [WIND_R4__Q_PCC] -> ResourceStatusBus/2  "Q_var"
  [WIND_R4__Vdc_Meas] -> Health/1, DC Energy pu/1, ResourceStatusBus/9  "Vdc_V"
  [WIND_R4__ID_REF_RESOURCE] -> Current References/1
  Current References/1 -> Limit Factor/1
  [WIND_R4__ENABLE] -> Online Headroom/2
  [WIND_R4__Vabc_PCC_Meas] -> Vll RMS/1
  Headroom/1 -> Online Headroom/1
  Generator Speed/1 -> MSC Available Power/1(In1)
  [WIND_R4__OMEGA_RESOURCE] -> Frequency Hz/1
  [WIND_R4__P_PCC] -> ResourceStatusBus/1  "P_W"
  [WIND_R4__IQ_REF_RESOURCE] -> Current References/2
  Health/1 -> ResourceStatusBus/11  "healthy"
  Power Headroom Inputs/1 -> Headroom/1
  Frequency Hz/1 -> ResourceStatusBus/4  "frequency_Hz"
  MSC Available Power/1(available_power_W) -> Power Headroom Inputs/1, ResourceStatusBus/5
  Actual MSC Power/1 -> Power Headroom Inputs/2

== system GRID_SUPPORTED_WIND_R1/Wind Resource/02 PMSG dq Machine and Average MSC/01 Torque and Current References ==
  omega_g : Inport
  Dispatch Torque Limit : Subsystem
  MPPT Torque Reference : Fcn  Expr=0.5*(Wind.Kopt_Nm_per_rad_s2*u^2+PMSG.torque_limit_Nm-abs(Wind.Kopt_Nm_per_rad_s2*u^2-PMSG.torque_limit_Nm))
  Torque to iq : Gain  Gain=-1/(1.5*PMSG.pole_pairs*PMSG.psi_f_Wb)
  id Reference : Constant  Value=0
  iq Limit : Saturate  UpperLimit=PMSG.current_limit_A  LowerLimit=-PMSG.current_limit_A
  id_ref : Outport
  iq_ref : Outport  Port=2
  wires:
  iq Limit/1 -> iq_ref/1
  omega_g/1 -> MPPT Torque Reference/1, Dispatch Torque Limit/1(In1)
  Torque to iq/1 -> iq Limit/1
  Dispatch Torque Limit/1(Out1) -> Torque to iq/1
  MPPT Torque Reference/1 -> Dispatch Torque Limit/2(In2)
  id Reference/1 -> id_ref/1

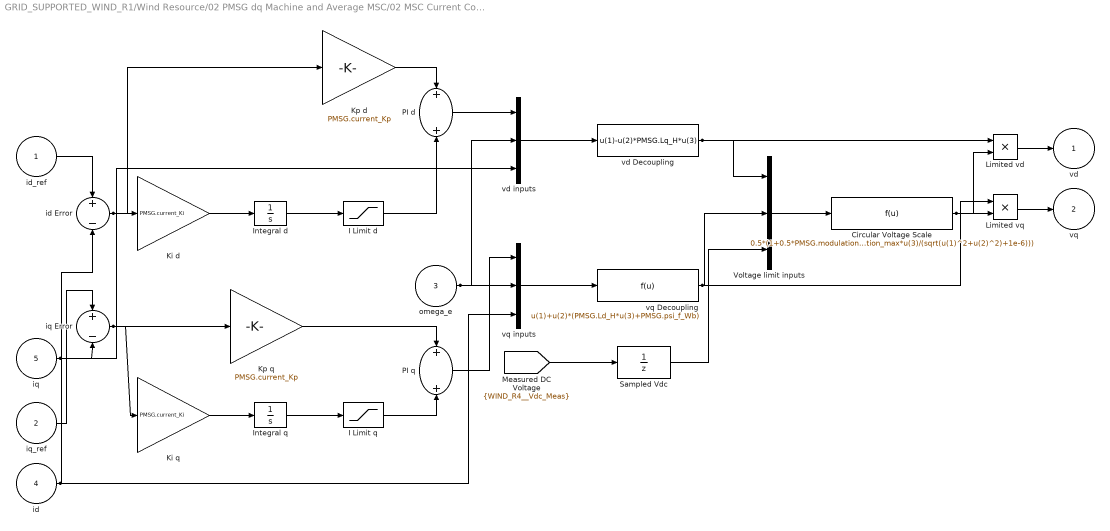
== system GRID_SUPPORTED_WIND_R1/Wind Resource/02 PMSG dq Machine and Average MSC/02 MSC Current Control ==
  id_ref : Inport
  iq_ref : Inport  Port=2
  omega_e : Inport  Port=3
  id : Inport  Port=4
  iq : Inport  Port=5
  Circular Voltage Scale : Fcn  Expr=0.5*(1+0.5*PMSG.modulation_max*u(3)/(sqrt(u(1)^2+u(2)^2)+1e-6)-abs(1-0.5*PMSG.modulation_max*u(3)/(sqrt(u(1)^2+u(2)^2)+1e-6)))
  I Limit d : Saturate  UpperLimit=PMSG.integrator_limit_V  LowerLimit=-PMSG.integrator_limit_V
  I Limit q : Saturate  UpperLimit=PMSG.integrator_limit_V  LowerLimit=-PMSG.integrator_limit_V
  Integral d : Integrator  InitialCondition=PMSG.Init.vd_pi_V
  Integral q : Integrator  InitialCondition=PMSG.Init.vq_pi_V
  Ki d : Gain  Gain=PMSG.current_Ki
  Ki q : Gain  Gain=PMSG.current_Ki
  Kp d : Gain  Gain=PMSG.current_Kp
  Kp q : Gain  Gain=PMSG.current_Kp
  Limited vd : Product
  Limited vq : Product
  PI d : Sum
  PI q : Sum
  Sampled Vdc : UnitDelay  InitialCondition=Converter.Vdc_nom  SampleTime=Control.Ts
  Voltage limit inputs : Mux  Inputs=3
  id Error : Sum  Inputs=+-
  iq Error : Sum  Inputs=+-
  vd Decoupling : Fcn  Expr=u(1)-u(2)*PMSG.Lq_H*u(3)
  vd inputs : Mux  Inputs=3
  vq Decoupling : Fcn  Expr=u(1)+u(2)*(PMSG.Ld_H*u(3)+PMSG.psi_f_Wb)
  vq inputs : Mux  Inputs=3
  vd : Outport
  vq : Outport  Port=2
  wires:
  iq/1 -> iq Error/2, vd inputs/3
  iq Error/1 -> Kp q/1, Ki q/1
  Ki d/1 -> Integral d/1
  vq Decoupling/1 -> Limited vq/1, Voltage limit inputs/2
  id Error/1 -> Kp d/1, Ki d/1
  iq_ref/1 -> iq Error/1
  PI q/1 -> vq inputs/1
  vd inputs/1 -> vd Decoupling/1
  id/1 -> id Error/2, vq inputs/3
  Ki q/1 -> Integral q/1
  id_ref/1 -> id Error/1
  Circular Voltage Scale/1 -> Limited vd/2, Limited vq/2
  Sampled Vdc/1 -> Voltage limit inputs/3
  Integral d/1 -> I Limit d/1
  Kp q/1 -> PI q/1
  [WIND_R4__Vdc_Meas] -> Sampled Vdc/1
  Integral q/1 -> I Limit q/1
  Kp d/1 -> PI d/1
  vq inputs/1 -> vq Decoupling/1
  I Limit d/1 -> PI d/2
  omega_e/1 -> vd inputs/2, vq inputs/2
  I Limit q/1 -> PI q/2
  PI d/1 -> vd inputs/1
  vd Decoupling/1 -> Limited vd/1, Voltage limit inputs/1
  Voltage limit inputs/1 -> Circular Voltage Scale/1
  Limited vd/1 -> vd/1
  Limited vq/1 -> vq/1

== system GRID_SUPPORTED_WIND_R1/Wind Resource/02 PMSG dq Machine and Average MSC/03 PMSG Electrical Dynamics ==
  vd : Inport
  vq : Inport  Port=2
  omega_e : Inport  Port=3
  Electromagnetic Torque : Fcn  Expr=-1.5*PMSG.pole_pairs*(PMSG.psi_f_Wb*u(2)+(PMSG.Ld_H-PMSG.Lq_H)*u(1)*u(2))
  Torque inputs : Mux  Inputs=2
  did dt : Fcn  Expr=(u(1)-PMSG.Rs_ohm*u(2)+u(3)*PMSG.Lq_H*u(4))/PMSG.Ld_H
  did inputs : Mux
  diq dt : Fcn  Expr=(u(1)-PMSG.Rs_ohm*u(2)-u(3)*(PMSG.Ld_H*u(4)+PMSG.psi_f_Wb))/PMSG.Lq_H
  diq inputs : Mux
  id State : Integrator  InitialCondition=PMSG.Init.id_A
  iq State : Integrator  InitialCondition=PMSG.Init.iq_A
  Te : Outport
  id : Outport  Port=2
  iq : Outport  Port=3
  wires:
  id State/1 -> diq inputs/4, Torque inputs/1, did inputs/2, id/1
  vd/1 -> did inputs/1
  diq inputs/1 -> diq dt/1
  Electromagnetic Torque/1 -> Te/1
  vq/1 -> diq inputs/1
  omega_e/1 -> did inputs/3, diq inputs/3
  did inputs/1 -> did dt/1
  iq State/1 -> did inputs/4, diq inputs/2, Torque inputs/2, iq/1
  diq dt/1 -> iq State/1
  Torque inputs/1 -> Electromagnetic Torque/1
  did dt/1 -> id State/1

== system GRID_SUPPORTED_WIND_R1/Wind Resource/02 PMSG dq Machine and Average MSC/04 MSC DC Power ==
  vd : Inport
  vq : Inport  Port=2
  id : Inport  Port=3
  iq : Inport  Port=4
  Generated DC Power : Fcn  Expr=-1.5*(u(1)*u(3)+u(2)*u(4))*PMSG.msc_efficiency-PMSG.loss_constant_W
  MSC Power Limit : Saturate  UpperLimit=PMSG.Sn_W  LowerLimit=0
  Power inputs : Mux
  Pdc : Outport
  wires:
  id/1 -> Power inputs/3
  vq/1 -> Power inputs/2
  vd/1 -> Power inputs/1
  Power inputs/1 -> Generated DC Power/1
  iq/1 -> Power inputs/4
  Generated DC Power/1 -> MSC Power Limit/1
  MSC Power Limit/1 -> Pdc/1

== system GRID_SUPPORTED_WIND_R1/Wind Resource/03 DC Link and Two-Level GSC/Converter AC Measurement ==
  note: VSC-side phase voltage, line voltage, and switching current are measured before the RL filter.
  Converter Terminal VI Sensor : ee_lib/Sensors & Transducers/Current and Voltage Sensor (Three-Phase)  port_option=ee.enum.threePhasePort.composite  vMeasurementType=ee.enum.vmeasurement.lg  outputUnit=ee.enum.unit.si  SRated=Base.Sn A*V  VRated=Base.Vll_lv V  I_specify=off  I_priority=None  I=[0, 0, 0] A  I_nominal_specify=off  I_nominal_value=1  I_nominal_unit=A  V_specify=off  V_priority=None  V=[0, 0, 0] V  V_nominal_specify=off  V_nominal_value=1  V_nominal_unit=V
  Iabc to Simulink : nesl_utility/PS-Simulink Converter  PhysicalDomain=network_engine_domain  SubClassName=ps_output  LeftPortType=input  RightPortType=output  PseudoPeriodic=off  Frequencies=[]  VectorFormat=inherit  Unit=A  AffineConversion=off
  Line Voltage Calculation : Subsystem
  Vabc to Simulink : nesl_utility/PS-Simulink Converter  PhysicalDomain=network_engine_domain  SubClassName=ps_output  LeftPortType=input  RightPortType=output  PseudoPeriodic=off  Frequencies=[]  VectorFormat=inherit  Unit=V  AffineConversion=off
  Vll Internal Monitor : Terminator
  From_VSC : PMIOPort  Side=Left
  To_Filter : PMIOPort  Port=2  Side=Right
  tag scope: WIND_R4__Iabc_Converter_Meas=scoped, WIND_R4__Vabc_Converter_Meas=scoped
  wires:
  Iabc to Simulink/1 -> [WIND_R4__Iabc_Converter_Meas]  "Iabc_Converter_Meas"
  Line Voltage Calculation/1(Vll) -> Vll Internal Monitor/1  "Vll_inv"
  Vabc to Simulink/1 -> [WIND_R4__Vabc_Converter_Meas], Line Voltage Calculation/1(Vabc)  "Vabc_Converter_Meas"
  connections:
  Converter Terminal VI Sensor/RConn2 -- Iabc to Simulink/LConn1
  Converter Terminal VI Sensor/RConn1 -- Vabc to Simulink/LConn1
  Converter Terminal VI Sensor/RConn3 -- To_Filter/RConn1
  From_VSC/RConn1 -- Converter Terminal VI Sensor/LConn1

== system GRID_SUPPORTED_WIND_R1/Wind Resource/03 DC Link and Two-Level GSC/DC Control and Monitoring ==
  note: MSC current command plus two explicit monitor outputs: sampled Vdc and estimated brake current.
  Vdc Measured : Inport
  Pmsc : Inport  Port=2
  Brake Current Estimate : Product
  Brake Current Limit : Saturate  UpperLimit=Wind.brake_current_limit_A  LowerLimit=0
  Brake Hysteresis : Relay  OnSwitchValue=Wind.brake_on_V  OffSwitchValue=Wind.brake_off_V
  Injection Sign : Gain
  MSC Current Inputs : Mux  Inputs=2
  MSC DC Current Limit : Saturate  UpperLimit=Wind.dc_current_limit_A  LowerLimit=0
  Net DC Injection : Sum  Inputs=+-
  P over Vdc : Fcn  Expr=2*u(1)/(u(2)+Wind.dc_voltage_floor_V+abs(u(2)-Wind.dc_voltage_floor_V))
  Sampled DC Voltage : UnitDelay  InitialCondition=Converter.Vdc_nom  SampleTime=Control.Ts
  Vdc over Brake R : Gain  Gain=1/Wind.brake_R_ohm
  I_msc Command : Outport
  Sampled Vdc : Outport  Port=2
  Brake Current : Outport  Port=3
  tag scope: WIND_R4__Vdc_Meas=scoped
  wires:
  Vdc over Brake R/1 -> Brake Current Estimate/2
  Brake Hysteresis/1 -> Brake Current Estimate/1
  Injection Sign/1 -> I_msc Command/1
  P over Vdc/1 -> MSC DC Current Limit/1
  MSC Current Inputs/1 -> P over Vdc/1
  Sampled DC Voltage/1 -> Sampled Vdc/1, MSC Current Inputs/2, Brake Hysteresis/1, Vdc over Brake R/1
  Vdc Measured/1 -> [WIND_R4__Vdc_Meas], Sampled DC Voltage/1
  Pmsc/1 -> MSC Current Inputs/1
  Brake Current Estimate/1 -> Brake Current Limit/1
  Brake Current Limit/1 -> Brake Current/1, Net DC Injection/2
  MSC DC Current Limit/1 -> Net DC Injection/1
  Net DC Injection/1 -> Injection Sign/1

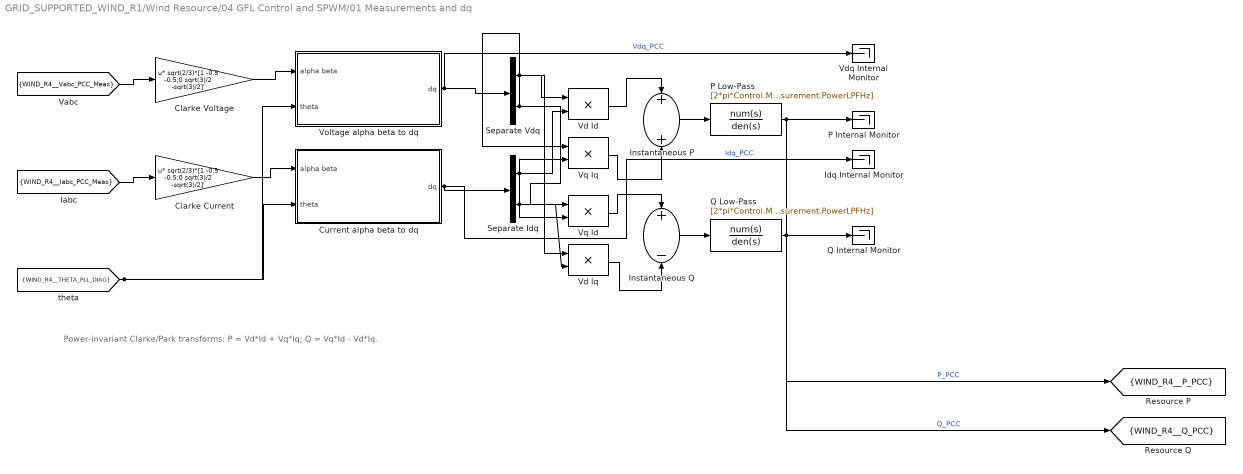
== system GRID_SUPPORTED_WIND_R1/Wind Resource/04 GFL Control and SPWM/01 Measurements and dq ==
  note: Power-invariant Clarke/Park transforms: P = Vd*Id + Vq*Iq; Q = Vq*Id - Vd*Iq.
  Clarke Current : Gain  Gain=sqrt(2/3)*[1 -0.5 -0.5;0 sqrt(3)/2 -sqrt(3)/2]'  Multiplication=Matrix(u*K)
  Clarke Voltage : Gain  Gain=sqrt(2/3)*[1 -0.5 -0.5;0 sqrt(3)/2 -sqrt(3)/2]'  Multiplication=Matrix(u*K)
  Current alpha beta to dq : Subsystem
  Idq Internal Monitor : Terminator
  Instantaneous P : Sum
  Instantaneous Q : Sum  Inputs=+-
  P Internal Monitor : Terminator
  P Low-Pass : TransferFcn  Numerator=[2*pi*Control.Measurement.PowerLPFHz]  Denominator=[1 2*pi*Control.Measurement.PowerLPFHz]
  Q Internal Monitor : Terminator
  Q Low-Pass : TransferFcn  Numerator=[2*pi*Control.Measurement.PowerLPFHz]  Denominator=[1 2*pi*Control.Measurement.PowerLPFHz]
  Separate Idq : Demux  Outputs=2
  Separate Vdq : Demux  Outputs=2
  Vd Id : Product
  Vd Iq : Product
  Vdq Internal Monitor : Terminator
  Voltage alpha beta to dq : Subsystem
  Vq Id : Product
  Vq Iq : Product
  tag scope: WIND_R4__P_PCC=scoped, WIND_R4__Q_PCC=scoped
  wires:
  Separate Vdq/2 -> Vq Iq/1, Vq Id/1
  Clarke Voltage/1 -> Voltage alpha beta to dq/1(alpha beta)
  Separate Idq/2 -> Vq Iq/2, Vd Iq/2
  Separate Idq/1 -> Vq Id/2, Vd Id/2
  Separate Vdq/1 -> Vd Iq/1, Vd Id/1
  Voltage alpha beta to dq/1(dq) -> Vdq Internal Monitor/1, Separate Vdq/1  "Vdq_PCC"
  Instantaneous Q/1 -> Q Low-Pass/1
  Q Low-Pass/1 -> Q Internal Monitor/1, [WIND_R4__Q_PCC]  "Q_PCC"
  Instantaneous P/1 -> P Low-Pass/1
  P Low-Pass/1 -> P Internal Monitor/1, [WIND_R4__P_PCC]  "P_PCC"
  Vd Iq/1 -> Instantaneous Q/2
  Vq Id/1 -> Instantaneous Q/1
  Vq Iq/1 -> Instantaneous P/2
  Vd Id/1 -> Instantaneous P/1
  Current alpha beta to dq/1(dq) -> Separate Idq/1, Idq Internal Monitor/1  "Idq_PCC"
  [WIND_R4__THETA_PLL_DIAG] -> Voltage alpha beta to dq/2(theta), Current alpha beta to dq/2(theta)
  Clarke Current/1 -> Current alpha beta to dq/1(alpha beta)
  [WIND_R4__Vabc_PCC_Meas] -> Clarke Voltage/1
  [WIND_R4__Iabc_PCC_Meas] -> Clarke Current/1

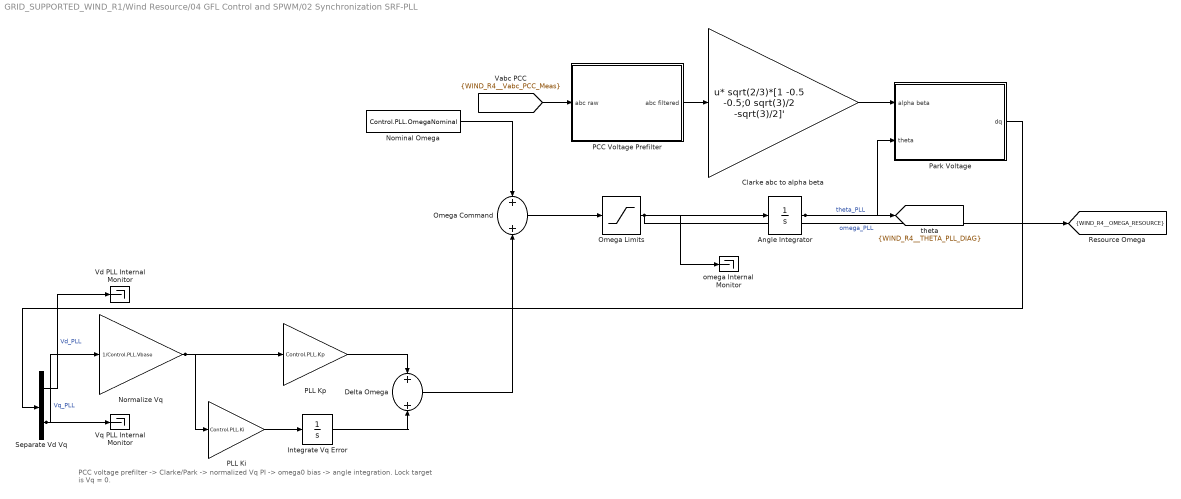
== system GRID_SUPPORTED_WIND_R1/Wind Resource/04 GFL Control and SPWM/02 Synchronization SRF-PLL ==
  note: PCC voltage prefilter -> Clarke/Park -> normalized Vq PI -> omega0 bias -> angle integration. Lock target is Vq = 0.
  Angle Integrator : Integrator  InitialCondition=Control.PLL.Theta0
  Clarke abc to alpha beta : Gain  Gain=sqrt(2/3)*[1 -0.5 -0.5;0 sqrt(3)/2 -sqrt(3)/2]'  Multiplication=Matrix(u*K)
  Delta Omega : Sum
  Integrate Vq Error : Integrator
  Nominal Omega : Constant  Value=Control.PLL.OmegaNominal
  Normalize Vq : Gain  Gain=1/Control.PLL.Vbase
  Omega Command : Sum
  Omega Limits : Saturate  UpperLimit=Control.PLL.OmegaMax  LowerLimit=Control.PLL.OmegaMin
  PCC Voltage Prefilter : Subsystem
  PLL Ki : Gain  Gain=Control.PLL.Ki
  PLL Kp : Gain  Gain=Control.PLL.Kp
  Park Voltage : Subsystem
  Separate Vd Vq : Demux  Outputs=2
  Vd PLL Internal Monitor : Terminator
  Vq PLL Internal Monitor : Terminator
  omega Internal Monitor : Terminator
  tag scope: WIND_R4__OMEGA_RESOURCE=scoped, WIND_R4__THETA_PLL_DIAG=scoped
  wires:
  Separate Vd Vq/2 -> Normalize Vq/1, Vq PLL Internal Monitor/1  "Vq_PLL"
  Omega Limits/1 -> Angle Integrator/1, omega Internal Monitor/1, [WIND_R4__OMEGA_RESOURCE]  "omega_PLL"
  PLL Kp/1 -> Delta Omega/1
  Normalize Vq/1 -> PLL Kp/1, PLL Ki/1
  PLL Ki/1 -> Integrate Vq Error/1
  Separate Vd Vq/1 -> Vd PLL Internal Monitor/1  "Vd_PLL"
  Integrate Vq Error/1 -> Delta Omega/2
  Nominal Omega/1 -> Omega Command/1
  [WIND_R4__Vabc_PCC_Meas] -> PCC Voltage Prefilter/1(abc raw)
  Delta Omega/1 -> Omega Command/2
  PCC Voltage Prefilter/1(abc filtered) -> Clarke abc to alpha beta/1
  Omega Command/1 -> Omega Limits/1
  Clarke abc to alpha beta/1 -> Park Voltage/1(alpha beta)
  Angle Integrator/1 -> Park Voltage/2(theta), [WIND_R4__THETA_PLL_DIAG]  "theta_PLL"
  Park Voltage/1(dq) -> Separate Vd Vq/1
